simulink library "Engine_Lib"  (R2025a)
settings: Solver=ode45  StartTime=0.0  StopTime=10.0  RelTol=1e-3  EnableMultiTasking=on
undefined symbols (not defined in the file or in its folder): AFR_Table, beta, center, coeffs, DCT_Param, ECP_Table, exponent, ICP_Table, invDG, Load_Table, numterms, polyTerms, S_Table, WendlandNumTerms, width
libraries: fl_lib x8, nesl_utility x6, sdl_lib x1
(part 1 of 2)
Description:
  | Copyright 2014-2025 The MathWorks, Inc.
settings Model: Creator=smiller  LastModifiedBy=smiller
settings SolverCC: AlgebraicLoopSolver=TrustRegion
settings DataIOCC: LimitDataPoints=on  SaveFormat=Array  SignalLoggingSaveFormat=ModelDataLogs  ReturnWorkspaceOutputs=off
settings OptimizationCC: ReuseModelBlockBuffer=off  ExpressionDepthLimit=2147483647.0  LifeSpan=inf
settings DebuggingCC: UnderspecifiedInitializationDetection=Classic  MergeDetectMultiDrivingBlocksExec=none  SolverPrmCheckMsg=warning  FcnCallInpInsideContextMsg=warning  UnconnectedInputMsg=warning  UnconnectedOutputMsg=warning  UnconnectedLineMsg=warning  AllowSymbolicDim=off  StateNameClashWarn=warning  PregeneratedLibrarySubsystemCodeDiagnostic=none  SFUnexpectedBacktrackingDiag=warning  SFNoUnconditionalDefaultTransitionDiag=warning  SFExecutionAtInitializationDiag=none  ArithmeticOperatorsInVariantConditions=warning
settings HardwareCC: ProdBitPerPointer=32.0  ProdBitPerSizeT=32.0  ProdBitPerPtrDiffT=32.0  ProdLargestAtomicFloat=None  ProdIntDivRoundTo=Undefined  ProdEndianess=Unspecified  ProdWordSize=32.0  ProdHWDeviceType=32-bit Generic
settings ModelReferenceCC: EnableRefExpFcnMdlSchedulingChecks=on  PropagateSignalLabelsOutOfModel=off
settings SFSimCC: SimUseLocalCustomCode=off  CustomCodeUndefinedFunction=UseInterfaceOnly
settings RTWCC: RTWUseLocalCustomCode=off  GPUComputeCapability=3.5  DLArmComputeVersion=19.05
settings CodeAppCC: StateflowObjectComments=on
settings GRTTargetCC: TargetLangStandard=C89/C90 (ANSI)  CombineOutputUpdateFcns=off  GRTInterface=on
settings ConfigComp: CovMetricSettings=dw  CovSaveCumulativeToWorkspaceVar=on  CovSaveSingleToWorkspaceVar=on  CovExternalEMLEnable=off  CovSFcnEnable=off

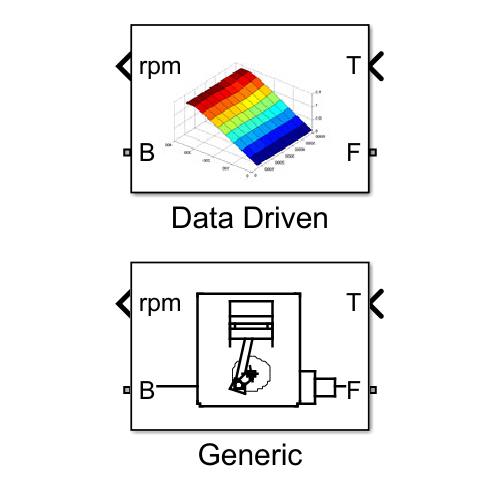
[thumbnail: Simulink's stored preview of the top-level diagram]
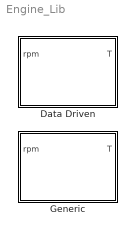
== system Engine_Lib ==
  Data Driven : Subsystem
      mask Display: image(imread('DCT_Engine_Data_Driven_IMAGE.jpg'));
  Generic : Subsystem
      mask Display:
      | plot([200.294537656123;201.704177092068;202.879954177142;203.81054553527;204.486989062962;204.902770239264;205.053884864158;204.938877621199;204.558856093007;203.917480094638;203.02092642757;201.877829393721;200.499197642409;198.898308151034;197.090578360535;195.093417696999;192.926059909376;191.349221415216], [79.0962651705123;81.4129472419303;83.856642682368;86.4038173688741;89.0299406167901;91.7097214236537;94.4173520353776;97.1267564890293;99.8118417386092;102.446748945347;105.006102512455;107.465254465996;109.80052182835;111.989414698229;114.010852840726;115.845368701499;117.475294889959;118.468271604945])
      | plot([180.070315486255;177.215173525063;174.340173090774;171.473002009205;168.641272705228;165.872256280019;163.192619875453;160.628169854943;158.203603274058;155.942270034374;153.865948011161;151.994633320535;150.346347745932;148.936965178479;147.780058742747;146.886770080143;146.265702048809;145.922835873396;145.861473542603;146.08220600922;146.58290749893;147.358755982674;148.402279615432;149.703428694174;151.249672441989;153.026119686324;155.015662269112;157.199139807684;159.555524219735;162.062122235246;164.694793945081;167.42818528151;170.23597219174;173.091114152932;175.966114587221;178.83328566879;181.665014972767;184.434031397976;185.486929355725], [123.25590763568;123.598773811093;123.660136141886;123.439403675268;122.938702185559;122.162853701815;121.119330069056;119.818180990315;118.2719372425;116.495489998164;114.505947415377;112.322469876805;109.966085464754;107.459487449243;104.826815739408;102.093424402979;99.2856374927491;96.4304955315569;93.5554950972677;90.688324015699;87.8565947117214;85.0875782865128;82.4079418819464;79.8434918614364;77.4189252805513;75.1575920408679;73.081270017655;71.2099553270291;69.5616697524256;68.1522871849724;66.9953807492411;66.1020920866371;65.4810240553025;65.1381578798894;65.0767955490969;65.2975280157144;65.7982295054238;66.5740779891678;66.9481130562871])
      | plot([182.088349247351;182.056804583223;181.962474383197;181.806267098667;181.589687091173;181.314820144583;180.98431337785;180.601349751811;180.169617415534;179.693274187426;179.176907513169;178.625490286111;178.044332955585;177.439032384376;176.815417947876;176.17949539401;175.537389004603;174.895282615196;174.25936006133;173.63574562483;173.030445053621;172.449287723095;171.897870496037;171.38150382178;170.905160593672;170.473428257395;170.090464631356;169.759957864623;169.485090918033;169.268510910539;169.112303626009;169.017973425983;168.986428761855;169.017973425983;169.112303626009;169.268510910539;169.485090918033;169.759957864623;170.090464631356;170.473428257395;170.905160593672;171.38150382178;171.897870496037;172.449287723095;173.030445053621;173.63574562483;174.25936006133;174.895282615196;175.537389004603;176.17949539401;176.815417947876;177.439032384376;178.044332955585;178.625490286111;179.176907513169;179.693274187426;180.169617415534;180.601349751811;180.98431337785;181.314820144583;181.589687091173;181.806267098667;181.962474383197;182.056804583223;182.088349247351;182.088349247351], [94.3432759959251;93.7073437064164;93.0775357924916;92.4599176486499;91.8604372752408;91.2848679959696;90.7387528576339;90.2273512475527;89.7555882427917;89.3280071789786;88.9487258954975;88.6213970784445;88.3491730832641;88.1346755758426;87.9799702844327;87.8865471055612;87.8553057555109;87.8865471055612;87.9799702844327;88.1346755758426;88.3491730832641;88.6213970784445;88.9487258954975;89.3280071789786;89.7555882427917;90.2273512475527;90.7387528576339;91.2848679959696;91.8604372752408;92.4599176486499;93.0775357924916;93.7073437064164;94.3432759959251;94.9792082854337;95.6090161993586;96.2266343432003;96.8261147166093;97.4016839958805;97.9477991342162;98.4592007442974;98.9309637490584;99.3585448128716;99.7378260963527;100.065154913406;100.337378908586;100.551876416008;100.706581707417;100.800004886289;100.831246236339;100.800004886289;100.706581707417;100.551876416008;100.337378908586;100.065154913406;99.7378260963526;99.3585448128716;98.9309637490584;98.4592007442974;97.9477991342162;97.4016839958805;96.8261147166093;96.2266343432003;95.6090161993586;94.9792082854338;94.3432759959251;94.3432759959251])
      | plot([201.615249970928;201.583705306799;201.489375106774;201.333167822243;201.11658781475;200.84172086816;200.511214101427;200.128250475388;199.69651813911;199.220174911002;198.703808236745;198.152391009688;197.571233679162;196.965933107953;196.342318671452;195.706396117586;195.06428972818;194.422183338773;193.786260784907;193.162646348407;192.557345777197;191.976188446671;191.424771219614;190.908404545357;190.432061317249;190.000328980971;189.617365354932;189.286858588199;189.011991641609;188.795411634116;188.639204349585;188.54487414956;188.513329485431;188.54487414956;188.639204349585;188.795411634116;189.011991641609;189.286858588199;189.617365354932;190.000328980971;190.432061317249;190.908404545357;191.424771219614;191.976188446671;192.557345777197;193.162646348407;193.786260784907;194.422183338773;195.06428972818;195.706396117586;196.342318671452;196.965933107953;197.571233679162;198.152391009688;198.703808236745;199.220174911002;199.69651813911;200.128250475388;200.511214101427;200.84172086816;201.11658781475;201.333167822243;201.489375106774;201.583705306799;201.615249970928;201.615249970928], [74.7533852700144;74.1174529805057;73.487645066581;72.8700269227392;72.2705465493302;71.694977270059;71.1488621317233;70.6374605216421;70.165697516881;69.7381164530679;69.3588351695868;69.0315063525339;68.7592823573535;68.5447848499319;68.390079558522;68.2966563796505;68.2654150296003;68.2966563796505;68.390079558522;68.5447848499319;68.7592823573535;69.0315063525339;69.3588351695868;69.7381164530679;70.165697516881;70.6374605216421;71.1488621317233;71.694977270059;72.2705465493302;72.8700269227392;73.487645066581;74.1174529805057;74.7533852700144;75.3893175595231;76.0191254734479;76.6367436172896;77.2362239906986;77.8117932699698;78.3579084083055;78.8693100183867;79.3410730231478;79.7686540869609;80.147935370442;80.4752641874949;80.7474881826754;80.9619856900969;81.1166909815068;81.2101141603783;81.2413555104285;81.2101141603783;81.1166909815068;80.9619856900969;80.7474881826753;80.4752641874949;80.147935370442;79.7686540869609;79.3410730231478;78.8693100183867;78.3579084083055;77.8117932699698;77.2362239906986;76.6367436172896;76.0191254734479;75.3893175595231;74.7533852700145;74.7533852700144])
      | plot([201.615249970928;201.583705306799;201.489375106774;201.333167822243;201.11658781475;200.84172086816;200.511214101427;200.128250475388;199.69651813911;199.220174911002;198.703808236745;198.152391009688;197.571233679162;196.965933107953;196.342318671452;195.706396117586;195.06428972818;194.422183338773;193.786260784907;193.162646348407;192.557345777197;191.976188446671;191.424771219614;190.908404545357;190.432061317249;190.000328980971;189.617365354932;189.286858588199;189.011991641609;188.795411634116;188.639204349585;188.54487414956;188.513329485431;188.54487414956;188.639204349585;188.795411634116;189.011991641609;189.286858588199;189.617365354932;190.000328980971;190.432061317249;190.908404545357;191.424771219614;191.976188446671;192.557345777197;193.162646348407;193.786260784907;194.422183338773;195.06428972818;195.706396117586;196.342318671452;196.965933107953;197.571233679162;198.152391009688;198.703808236745;199.220174911002;199.69651813911;200.128250475388;200.511214101427;200.84172086816;201.11658781475;201.333167822243;201.489375106774;201.583705306799;201.615249970928;201.615249970928], [74.7533852700144;74.1174529805057;73.487645066581;72.8700269227392;72.2705465493302;71.694977270059;71.1488621317233;70.6374605216421;70.165697516881;69.7381164530679;69.3588351695868;69.0315063525339;68.7592823573535;68.5447848499319;68.390079558522;68.2966563796505;68.2654150296003;68.2966563796505;68.390079558522;68.5447848499319;68.7592823573535;69.0315063525339;69.3588351695868;69.7381164530679;70.165697516881;70.6374605216421;71.1488621317233;71.694977270059;72.2705465493302;72.8700269227392;73.487645066581;74.1174529805057;74.7533852700144;75.3893175595231;76.0191254734479;76.6367436172896;77.2362239906986;77.8117932699698;78.3579084083055;78.8693100183867;79.3410730231478;79.7686540869609;80.147935370442;80.4752641874949;80.7474881826754;80.9619856900969;81.1166909815068;81.2101141603783;81.2413555104285;81.2101141603783;81.1166909815068;80.9619856900969;80.7474881826753;80.4752641874949;80.147935370442;79.7686540869609;79.3410730231478;78.8693100183867;78.3579084083055;77.8117932699698;77.2362239906986;76.6367436172896;76.0191254734479;75.3893175595231;74.7533852700145;74.7533852700144])
      | plot([142.90856779553;142.90856779553;208.103220211342;208.103220211342], [139.948037685826;218.181620584801;218.181620584801;139.948037685826])
      | plot([142.90856779553;208.103220211342], [179.064829135314;179.064829135314])
      | plot([149.459528038278;149.459528038278], [179.064829135314;172.576858894899])
      | plot([201.615249970928;201.615249970928], [179.064829135314;172.576858894899])
      | plot([142.90856779553;208.103220211342;208.103220211342;142.90856779553;142.90856779553], [179.064829135314;179.064829135314;152.986968168989;152.986968168989;179.064829135314])
      | plot([142.90856779553;208.103220211342], [192.103759618476;192.103759618476])
      | plot([180.639579193667;200.229469919577], [99.0045361686498;79.4776354450732])
      | plot([173.332738922909;192.92262964882], [87.8553057555109;68.3284050319344])
      | plot([183.663099305704;200.481429928914], [153.553878189996;76.9580353517085])
      | plot([184.544959338382;174.970478983596], [95.0361660216004;153.553878189996])
      | plot([183.474129298702;186.749609420076;206.654450157657;201.615249970928;197.961829835549], [76.9580353517085;62.0923948008567;67.8874750155956;88.1702557671815;87.7923157531768])
      | plot([164.199188584462;187.694459455088], [94.7842060122639;95.1621460262686])
      | plot([175.537389004603;175.285428995267], [106.50034644641;81.9342455361038])
      | plot([142.90856779553;208.103220211342], [172.576858894899;172.576858894899])
      | plot([255.86397353746;317.389525743201], [71.0999651346356;71.0999651346356])
      | plot([80.518472487107;50.86397353746;50.86397353746;80.518472487107;80.518472487107], [85.2727156598121;85.2727156598121;56.927214609459;56.927214609459;85.2727156598121])
      | plot([102.180272066966;80.518472487107;80.518472487107;102.180272066966], [42.7544640842825;42.7544640842825;99.4454661849886;99.4454661849886])
      | plot([108.893966535106;108.245686045801;107.603648851995;106.974038122836;106.362917353826;105.776171972045;105.219452656266;104.698120917834;104.217197466378;103.781313857637;103.394667889039;103.060983172626;102.783473274627;102.564810767061;102.40710148941;102.31186426823;102.280016290024;102.280016290024;102.31186426823;102.40710148941;102.564810767061;102.783473274627;103.060983172626;103.394667889039;103.781313857637;104.217197466378;104.698120917834;105.219452656266;105.776171972045;106.362917353826;106.974038122836;107.603648851995;108.245686045801;108.893966535106;249.67662175186;250.324902241165;250.966939434972;251.596550164131;252.20767093314;252.794416314921;253.3511356307;253.872467369133;254.353390820588;254.78927442933;255.175920397927;255.50960511434;255.787115012339;256.005777519905;256.163486797556;256.258724018736;256.290571996942;256.290571996942;256.258724018736;256.163486797556;256.005777519905;255.787115012339;255.50960511434;255.175920397927;254.78927442933;254.353390820588;253.872467369133;253.3511356307;252.794416314921;252.20767093314;251.596550164131;250.966939434972;250.324902241165;249.67662175186;108.893966535106], [233.173241140321;233.141393162114;233.046155940935;232.888446663284;232.669784155718;232.392274257719;232.058589541306;231.671943572708;231.236059963967;230.755136512511;230.233804774079;229.6770854583;229.090340076519;228.479219307509;227.84960857835;227.207571384544;226.559290895239;46.5338642243296;45.8855837350246;45.2435465412178;44.6139358120588;44.0028150430496;43.4160696612682;42.8593503454891;42.3380186070568;41.8570951556014;41.4212115468599;41.0345655782626;40.7008808618494;40.42337096385;40.2047084562844;40.0469991786335;39.9517619574538;39.9199139792472;39.9199139792472;39.9517619574538;40.0469991786335;40.2047084562844;40.42337096385;40.7008808618494;41.0345655782626;41.4212115468599;41.8570951556014;42.3380186070568;42.8593503454891;43.4160696612682;44.0028150430496;44.6139358120588;45.2435465412178;45.8855837350246;46.5338642243296;226.559290895239;227.207571384544;227.84960857835;228.479219307509;229.090340076519;229.6770854583;230.233804774079;230.755136512511;231.236059963967;231.671943572708;232.058589541306;232.392274257719;232.669784155718;232.888446663284;233.046155940935;233.141393162114;233.173241140321;233.173241140321])
      | plot([50.280016290024;35.236212508752942], [71.0999651346356;71.0999651346356]);
      | patch([0;354.791188146919;354.791188146919;0;0;0.472425017505884;0.472425017505884;354.318763129413;354.318763129413;0.472425017505884;0], [283.927435521036;283.927435521036;0;0;283.927435521036;283.455010503531;0.472425017505884;0.472425017505884;283.455010503531;283.455010503531;283.927435521036], [1;1;1])

== system Engine_Lib/Data Driven ==
  T : Inport
  Engine Control Software : Subsystem
  Inertia : fl_lib/Mechanical/Rotational Elements/Inertia  inertia=DCT_Param.ICE.Shaft_Inertia kg*m^2  num_ports=foundation.enum.numPorts2.one  w_specify=on  w_priority=High  w=DCT_Param.ICE.Initial_Velocity rpm  w_nominal_specify=off  w_nominal_value=1  w_nominal_unit=rad/s  t_specify=off  t_priority=High  t=0 N*m  t_nominal_specify=off  t_nominal_value=1  t_nominal_unit=N*m
  MBC Engine Model From Dynamometer Data : Subsystem
      mask Display:
      | image(imread('DCT_Engine_Data_Driven_IMAGE.jpg'),'center')
      | port_label('input',1,'Bus')
      | port_label('output',1,'rpm')
      | color('red');
      | port_label('LConn',1,'B')
      | port_label('RConn',1,'F')
  B : PMIOPort  Side=Right
  F : PMIOPort  Port=2  Side=Left
  rpm : Outport  VectorParamsAs1DForOutWhenUnconnected=off
  wires:
  Engine Control Software/1(Engine Control Bus) -> MBC Engine Model From Dynamometer Data/1(Engine Control Bus)
  MBC Engine Model From Dynamometer Data/1(Engine Speed) -> Engine Control Software/1(Engine Speed), rpm/1
  T/1 -> Engine Control Software/2(Torque Demand)
  connections:
  B/RConn1 -- MBC Engine Model From Dynamometer Data/LConn1
  F/RConn1 -- MBC Engine Model From Dynamometer Data/RConn1 -- Inertia/LConn1

== system Engine_Lib/Generic ==
  T : Inport
  Engine Management : Subsystem
  Fuel Consumption : Subsystem
  Generic Engine : sdl_lib/Engines & Motors/Generic Engine  input_type=sdl.enum.GenericEngineInputType.NormalizedThrottle  model_parameterization=1  engine_type=1  Trq_max=380 N*m  w_Trq_max=4300 rpm  P_max=DCT_Param.ICE.Max_Power W  w_P_max=DCT_Param.ICE.Speed_At_Max_Power rpm  w_max=DCT_Param.ICE.Max_Speed rpm  w_min=DCT_Param.ICE.Stall_Speed rpm  w_tab=[ 500 1000 2e+3 3e+3 4e+3 5e+3 6e+3 7e+3 ] rpm  trq_tab=[ 380 380 380 380 350 280 200 80 ] N*m  pwr_tab=[ 2e+4 4e+4 7.8e+4 1.2e+5 1.45e+5 1.48e+5 1.25e+5 6e+4 ] W  interp_method=1  w_thr=DCT_Param.ICE.Speed_Threshold rpm  model_inertia=1  inertia=DCT_Param.ICE.Shaft_Inertia kg*m^2  initial_velocity=DCT_Param.ICE.Initial_Velocity rpm  model_time_constant=1  time_constant=DCT_Param.ICE.Engine_Time_Constant s  initial_normalized_throttle=DCT_Param.ICE.Initial_Normalized_Throttle  fc_model=1  fc_per_rev=25 mg/rev  fc_w_tab=[ 1000 2e+3 3e+3 4e+3 5e+3 6e+3 ] rpm  fc_trq_tab=[ 0 80 160 200 240 320 360 400 ] N*m  fc_tab=[ 0.5 0.9 1.4 1.6 1.9 2.7 3.4 4.4; 1 1.7 2.7 3.1 3.6 5 6 7.4; 1.4 2.7 4 4.8 5.6 7.5 8.5 10.5; 2 3.6 5.8 6.7 8 10.4 11.7 13.3; 2.5 4.8 7.9 9.4 10.8 14 16.2 18.6; 3.1 6 10.3 11.9 13.8 18.4 22 26.5 ] g/s  bmep_tab=[ 0 250 500 625 750 1000 1.15e+3 1.25e+3 ] kPa  bsfc_tab=[ 410 380 300 280 270 290 320 380; 410 370 290 270 260 270 285 320; 415 380 290 275 265 270 270 300; 420 390 310 290 285 280 280 285; 430 410 340 320 310 300 310 320; 450 430 370 340 330 330 350 380 ] g/hr/kW  fc_interp_method=1  displaced_volume=400 cm^3  rev_per_cycle=2  idle_speed=0  idle_speed_reference=1000 rpm  tau_controller=1 s  idle_w_thr=1 rpm  redline=0  redline_speed=5000 rpm  tau_redline=1 s  redline_w_thr=1 rpm
      settings: InternalSimscapePortConfiguration="{\"Bottom\":[],\"Left\":[{\"id\":\"ThrNorm\",\"label\":\"Thr\",\"type\":\"input\"},{\"id\":\"B\",\"label\":\"B\",\"type\":\"foundation.mechanical.rotational.rotational\"}],\"Right\":[{\"id\":\"P\",\"label\":\"P\",\"type\":\"output\"},{\"id\":\"FC\",\"label\":\"FC\",\"type\":\"output\"},{\"id\":\"F\",\"label\":\"F\",\"type\":\"foundation.mechanical.rotational.rotational\"}],\"Top\":[]}"
  F : PMIOPort  Side=Left
  B : PMIOPort  Port=2  Side=Right
  rpm : Outport  VectorParamsAs1DForOutWhenUnconnected=off
  wires:
  T/1 -> Engine Management/2(TrqDem)
  Fuel Consumption/1(rpm) -> rpm/1, Engine Management/1(EngSpd)
  connections:
  B/RConn1 -- Generic Engine/LConn2
  Engine Management/RConn1 -- Generic Engine/LConn1
  Generic Engine/RConn3 -- Fuel Consumption/LConn1
  Fuel Consumption/RConn1 -- F/RConn1

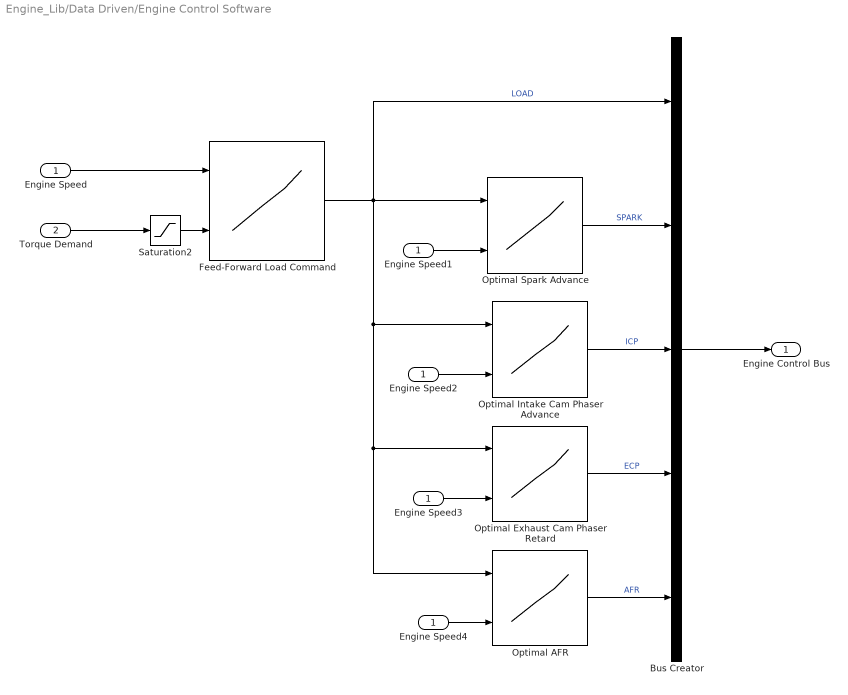
== system Engine_Lib/Data Driven/Engine Control Software ==
  Engine Speed : Inport
  Torque Demand : Inport  Port=2
  Bus Creator : BusCreator  Inputs=5
  Engine Speed{1..4} (4 alike) : InportShadow
  Feed-Forward Load Command : Lookup2D  RowIndex=Load_Table.Y  ColumnIndex=Load_Table.X  Table=Load_Table.Z  LookUpMeth=Interpolation-Use End Values  SaturateOnIntegerOverflow=off  InputSameDT=off
  Optimal AFR : Lookup2D  RowIndex=AFR_Table.Y  ColumnIndex=AFR_Table.X  Table=AFR_Table.Z  LookUpMeth=Interpolation-Use End Values  SaturateOnIntegerOverflow=off  InputSameDT=off
  Optimal Exhaust Cam Phaser Retard : Lookup2D  RowIndex=ECP_Table.Y  ColumnIndex=ECP_Table.X  Table=ECP_Table.Z  LookUpMeth=Interpolation-Use End Values  SaturateOnIntegerOverflow=off  InputSameDT=off
  Optimal Intake Cam Phaser Advance : Lookup2D  RowIndex=ICP_Table.Y  ColumnIndex=ICP_Table.X  Table=ICP_Table.Z  LookUpMeth=Interpolation-Use End Values  SaturateOnIntegerOverflow=off  InputSameDT=off
  Optimal Spark Advance : Lookup2D  RowIndex=S_Table.Y  ColumnIndex=S_Table.X  Table=S_Table.Z  LookUpMeth=Interpolation-Use End Values  SaturateOnIntegerOverflow=off  InputSameDT=off
  Saturation2 : Saturate  UpperLimit=inf  LowerLimit=0
  Engine Control Bus : Outport  VectorParamsAs1DForOutWhenUnconnected=off
  wires:
  Torque Demand/1 -> Saturation2/1
  Engine Speed/1 -> Feed-Forward Load Command/1
  Optimal Spark Advance/1 -> Bus Creator/2  "SPARK"
  Optimal Intake Cam Phaser Advance/1 -> Bus Creator/3  "ICP"
  Optimal Exhaust Cam Phaser Retard/1 -> Bus Creator/4  "ECP"
  Optimal AFR/1 -> Bus Creator/5  "AFR"
  Bus Creator/1 -> Engine Control Bus/1
  Engine Speed4/1 -> Optimal AFR/2
  Engine Speed3/1 -> Optimal Exhaust Cam Phaser Retard/2
  Engine Speed2/1 -> Optimal Intake Cam Phaser Advance/2
  Engine Speed1/1 -> Optimal Spark Advance/2
  Feed-Forward Load Command/1 -> Optimal Spark Advance/1, Optimal Intake Cam Phaser Advance/1, Optimal Exhaust Cam Phaser Retard/1, Optimal AFR/1, Bus Creator/1  "LOAD"
  Saturation2/1 -> Feed-Forward Load Command/2

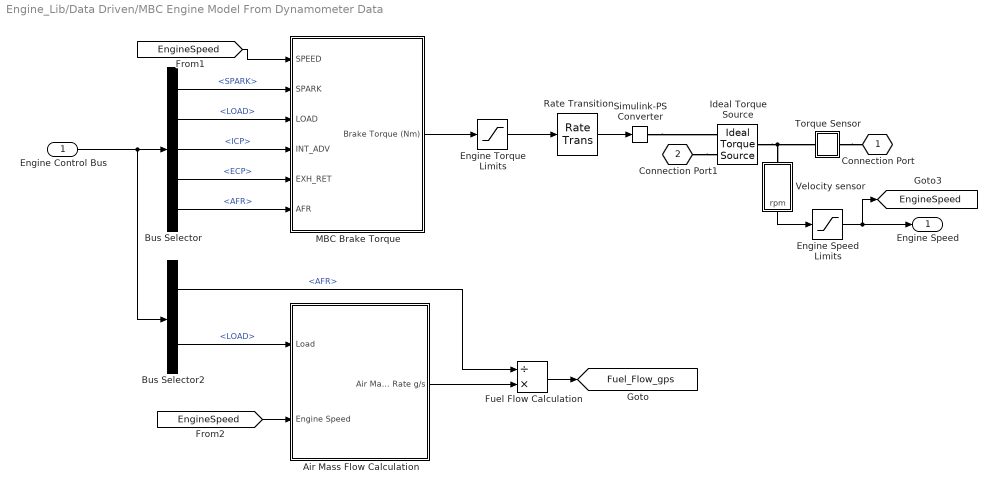
== system Engine_Lib/Data Driven/MBC Engine Model From Dynamometer Data ==
  Engine Control Bus : Inport
  Air Mass Flow Calculation : Subsystem
  Bus Selector : BusSelector  OutputSignals=SPARK,LOAD,ICP,ECP,AFR
  Bus Selector2 : BusSelector  OutputSignals=AFR,LOAD
  Engine Speed Limits : Saturate  UpperLimit=inf  LowerLimit=500
  Engine Torque Limits : Saturate  UpperLimit=Inf  LowerLimit=0.1
  Fuel Flow Calculation : Product  Inputs=/*  RndMeth=Zero
  Ideal Torque Source : fl_lib/Mechanical/Mechanical Sources/Ideal Torque Source
  MBC Brake Torque : Subsystem
  Rate Transition : RateTransition
  Simulink-PS Converter : nesl_utility/Simulink-PS Converter  PhysicalDomain=network_engine_domain  SubClassName=ps_input  LeftPortType=input  RightPortType=output  PseudoPeriodic=off  Frequencies=[]  NoiseDistribution=none  NoiseParameters=[]  Unit=1  AffineConversion=off  FilteringAndDerivatives=zero  SimscapeFilterOrder=1  InputFilterTimeConstant=0.005  UdotUserProvided=0
  Torque Sensor : Subsystem
      mask Display: disp('S')
  Velocity sensor : Subsystem
  Connection Port : PMIOPort  Side=Right
  Connection Port1 : PMIOPort  Port=2  Side=Left
  Engine Speed : Outport  VectorParamsAs1DForOutWhenUnconnected=off
  tag scope: EngineSpeed=global, Fuel_Flow_gps=global
  wires:
  Engine Torque Limits/1 -> Rate Transition/1
  Bus Selector2/2 -> Air Mass Flow Calculation/1(Load)  "<LOAD>"
  Bus Selector2/1 -> Fuel Flow Calculation/1  "<AFR>"
  Air Mass Flow Calculation/1(Air Mass Flow Rate g/s) -> Fuel Flow Calculation/2
  [EngineSpeed] -> Air Mass Flow Calculation/2(Engine Speed)
  Fuel Flow Calculation/1 -> [Fuel_Flow_gps]
  MBC Brake Torque/1(Brake Torque (Nm)) -> Engine Torque Limits/1
  Engine Control Bus/1 -> Bus Selector2/1, Bus Selector/1
  Rate Transition/1 -> Simulink-PS Converter/1
  Velocity sensor/1(rpm) -> Engine Speed Limits/1
  Engine Speed Limits/1 -> Engine Speed/1, [EngineSpeed]
  [EngineSpeed] -> MBC Brake Torque/1(SPEED)
  Bus Selector/1 -> MBC Brake Torque/2(SPARK)  "<SPARK>"
  Bus Selector/2 -> MBC Brake Torque/3(LOAD)  "<LOAD>"
  Bus Selector/3 -> MBC Brake Torque/4(INT_ADV)  "<ICP>"
  Bus Selector/4 -> MBC Brake Torque/5(EXH_RET)  "<ECP>"
  Bus Selector/5 -> MBC Brake Torque/6(AFR)  "<AFR>"
  connections:
  Ideal Torque Source/LConn1 -- Velocity sensor/LConn1 -- Torque Sensor/LConn1
  Connection Port1/RConn1 -- Ideal Torque Source/RConn2
  Simulink-PS Converter/RConn1 -- Ideal Torque Source/RConn1
  Torque Sensor/RConn1 -- Connection Port/RConn1

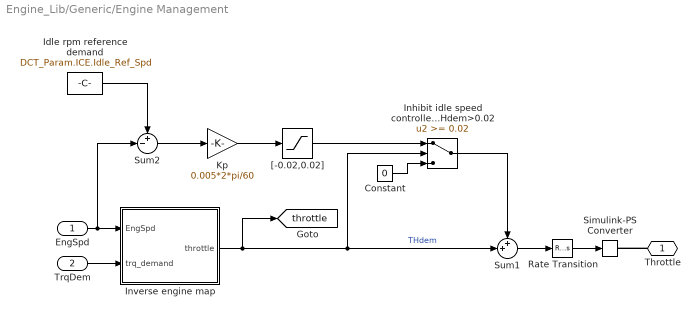
== system Engine_Lib/Generic/Engine Management ==
  EngSpd : Inport
  TrqDem : Inport  Port=2
  Constant : Constant  Value=0  SampleTime=0.01
  Idle rpm reference demand : Constant  Value=DCT_Param.ICE.Idle_Ref_Spd  SampleTime=0.01
  Inhibit idle speed controller if THdem>0.02 : Switch  Threshold=0.02  SaturateOnIntegerOverflow=off
  Inverse engine map : Subsystem  mask(Inverse engine map){P0=92000, rpm0=5500}
      mask prompts: P0 "Engine maximum power (W)"; rpm0 "Speed at maximum power (rpm)"
      mask help: Converts measured speed and demanded torque into normalized throttle demand. Assumes that the engine is modeled using the Simscape Driveline Generic Engine block with model parameterization set to Normalized 3rd-order polynomial matched to peak power.
      mask init:
      | w0 = 2*pi*rpm0/60;
  Kp : Gain  Gain=0.005*2*pi/60  SaturateOnIntegerOverflow=on  OutDataTypeStr=Inherit: Same as input  ParamDataTypeStr=Inherit: Same as input
  Rate Transition : RateTransition
  Simulink-PS Converter : nesl_utility/Simulink-PS Converter  PhysicalDomain=network_engine_domain  SubClassName=ps_input  LeftPortType=input  RightPortType=output  PseudoPeriodic=off  Frequencies=[]  NoiseDistribution=none  NoiseParameters=[]  Unit=1  AffineConversion=off  FilteringAndDerivatives=zero  SimscapeFilterOrder=1  InputFilterTimeConstant=0.005  UdotUserProvided=0
  Sum1 : Sum  Inputs=++|  InputSameDT=on  SaturateOnIntegerOverflow=on  OutDataTypeStr=Inherit: Same as first input
  Sum2 : Sum  Inputs=+-|  InputSameDT=on  SaturateOnIntegerOverflow=on  OutDataTypeStr=Inherit: Same as first input
  "[-0.02,0.02]" : Saturate  UpperLimit=0.02  LowerLimit=-0.02
  Throttle : PMIOPort  Side=Right
  tag scope: throttle=global
  wires:
  "[-0.02,0.02]"/1 -> Inhibit idle speed controller if THdem>0.02/1
  Kp/1 -> "[-0.02,0.02]"/1
  Sum2/1 -> Kp/1
  Idle rpm reference demand/1 -> Sum2/1
  Sum1/1 -> Rate Transition/1
  Constant/1 -> Inhibit idle speed controller if THdem>0.02/3
  Inhibit idle speed controller if THdem>0.02/1 -> Sum1/1
  EngSpd/1 -> Sum2/2, Inverse engine map/1(EngSpd)
  TrqDem/1 -> Inverse engine map/2(trq_demand)
  Inverse engine map/1(throttle) -> Inhibit idle speed controller if THdem>0.02/2, Sum1/2, [throttle]  "THdem"
  Rate Transition/1 -> Simulink-PS Converter/1
  connections:
  Throttle/RConn1 -- Simulink-PS Converter/RConn1

== system Engine_Lib/Generic/Fuel Consumption ==
  Filter : TransferFcn  Denominator=[DCT_Param.Transmission.Abstract.Ratio_Time_Const*2 1]
  Fuel Consumption Table : Lookup2D  RowIndex=DCT_Param.ICE.FC.Speed_Vector  ColumnIndex=DCT_Param.ICE.FC.Torque_Vector  Table=DCT_Param.ICE.FC.Consumption_Table  SaturateOnIntegerOverflow=off  InputSameDT=off
  Min of table : Saturate  UpperLimit=Inf  LowerLimit=min(min(DCT_Param.ICE.FC.Consumption_Table))
  Torque Sensor : Subsystem
      mask Display: disp('S')
  Velocity sensor : Subsystem
      mask Display: disp('S')
  B : PMIOPort  Side=Left
  F : PMIOPort  Port=2  Side=Right
  rpm : Outport  VectorParamsAs1DForOutWhenUnconnected=off
  tag scope: Fuel_Flow_gps=global
  wires:
  Velocity sensor/1(rpm) -> rpm/1, Fuel Consumption Table/1
  Fuel Consumption Table/1 -> Min of table/1
  Torque Sensor/1(rpm) -> Filter/1
  Filter/1 -> Fuel Consumption Table/2
  Min of table/1 -> [Fuel_Flow_gps]
  connections:
  B/RConn1 -- Torque Sensor/LConn1 -- Velocity sensor/LConn1
  Torque Sensor/RConn1 -- F/RConn1

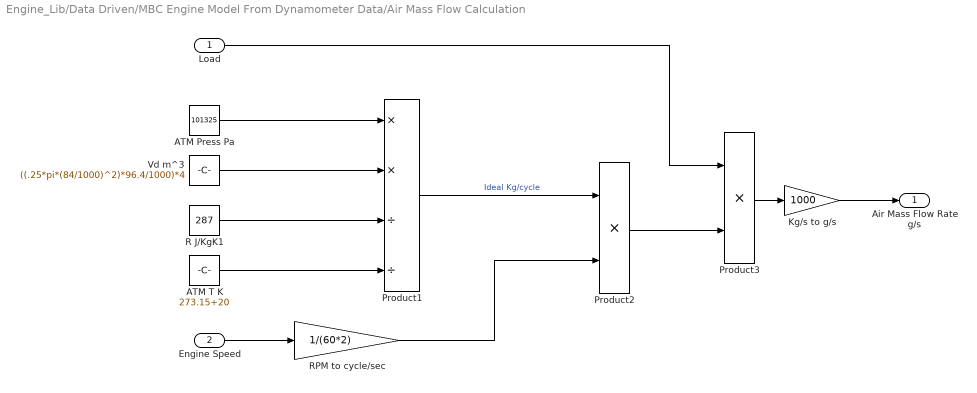
== system Engine_Lib/Data Driven/MBC Engine Model From Dynamometer Data/Air Mass Flow Calculation ==
  Load : Inport
  Engine Speed : Inport  Port=2
  ATM Press Pa : Constant  Value=101325
  ATM T K : Constant  Value=273.15+20
  Kg/s to g/s : Gain  Gain=1000
  Product1 : Product  Inputs=**//  InputSameDT=on  SaturateOnIntegerOverflow=on  OutDataTypeStr=Inherit: Same as first input
  Product2 : Product  Inputs=**  InputSameDT=on  SaturateOnIntegerOverflow=on  OutDataTypeStr=Inherit: Same as first input
  Product3 : Product  Inputs=**  InputSameDT=on  SaturateOnIntegerOverflow=on  OutDataTypeStr=Inherit: Same as first input
  R J/KgK1 : Constant  Value=287
  RPM to cycle/sec : Gain  Gain=1/(60*2)  SaturateOnIntegerOverflow=on  OutDataTypeStr=Inherit: Same as input  ParamDataTypeStr=Inherit: Same as input
  Vd m^3 : Constant  Value=((.25*pi*(84/1000)^2)*96.4/1000)*4
  Air Mass Flow Rate g/s : Outport  VectorParamsAs1DForOutWhenUnconnected=off
  wires:
  Kg/s to g/s/1 -> Air Mass Flow Rate g/s/1
  Product3/1 -> Kg/s to g/s/1
  Product2/1 -> Product3/2
  RPM to cycle/sec/1 -> Product2/2
  Engine Speed/1 -> RPM to cycle/sec/1
  Vd m^3/1 -> Product1/2
  ATM T K/1 -> Product1/4
  R J/KgK1/1 -> Product1/3
  ATM Press Pa/1 -> Product1/1
  Load/1 -> Product3/1
  Product1/1 -> Product2/1  "Ideal Kg/cycle"

== system Engine_Lib/Data Driven/MBC Engine Model From Dynamometer Data/MBC Brake Torque ==
  SPEED : Inport
  SPARK : Inport  Port=2
  LOAD : Inport  Port=3
  INT_ADV : Inport  Port=4
  EXH_RET : Inport  Port=5
  AFR : Inport  Port=6
  Mx1 : Mux  Inputs=6
  xregtwostage : Subsystem
  Brake Torque (Nm) : Outport  VectorParamsAs1DForOutWhenUnconnected=off
  wires:
  xregtwostage/1(Y) -> Brake Torque (Nm)/1
  Mx1/1 -> xregtwostage/1(X)
  AFR/1 -> Mx1/6
  EXH_RET/1 -> Mx1/5
  INT_ADV/1 -> Mx1/4
  LOAD/1 -> Mx1/3
  SPEED/1 -> Mx1/2
  SPARK/1 -> Mx1/1

== system Engine_Lib/Data Driven/MBC Engine Model From Dynamometer Data/Torque Sensor ==
  Ideal Torque Sensor : fl_lib/Mechanical/Mechanical Sensors/Ideal Torque Sensor
  PS-Simulink Converter1 : nesl_utility/PS-Simulink Converter  PhysicalDomain=network_engine_domain  SubClassName=ps_output  LeftPortType=input  RightPortType=output  PseudoPeriodic=off  Frequencies=[]  VectorFormat=1-D array  Unit=N*m  AffineConversion=off
  R : PMIOPort  Side=Left
  C : PMIOPort  Port=2  Side=Right
  tag scope: EngTrq_Nm=global
  wires:
  PS-Simulink Converter1/1 -> [EngTrq_Nm]
  connections:
  Ideal Torque Sensor/RConn2 -- PS-Simulink Converter1/LConn1
  C/RConn1 -- Ideal Torque Sensor/RConn1
  R/RConn1 -- Ideal Torque Sensor/LConn1

== system Engine_Lib/Data Driven/MBC Engine Model From Dynamometer Data/Velocity sensor ==
  Ideal Rotational Motion Sensor : fl_lib/Mechanical/Mechanical Sensors/Ideal Rotational Motion Sensor  reference=foundation.enum.MeasurementReference.difference  acceleration_port=false  velocity_port=true  position_port=true  wrap_angle=simscape.enum.onoff.off  offset=5 rad
  MRR : fl_lib/Mechanical/Rotational Elements/Mechanical Rotational Reference
  PS2S : nesl_utility/PS-Simulink Converter  PhysicalDomain=network_engine_domain  SubClassName=ps_output  LeftPortType=input  RightPortType=output  PseudoPeriodic=off  Frequencies=[]  VectorFormat=1-D array  Unit=rpm  AffineConversion=off
  Sensor dynamics : TransferFcn  Denominator=[0.01 1]
  Zero-Order Hold : ZeroOrderHold  SampleTime=0.01
  F : PMIOPort  Side=Left
  rpm : Outport  VectorParamsAs1DForOutWhenUnconnected=off
  wires:
  PS2S/1 -> Sensor dynamics/1
  Zero-Order Hold/1 -> rpm/1
  Sensor dynamics/1 -> Zero-Order Hold/1
  connections:
  F/RConn1 -- Ideal Rotational Motion Sensor/LConn1
  Ideal Rotational Motion Sensor/RConn2 -- PS2S/LConn1
  MRR/LConn1 -- Ideal Rotational Motion Sensor/RConn1

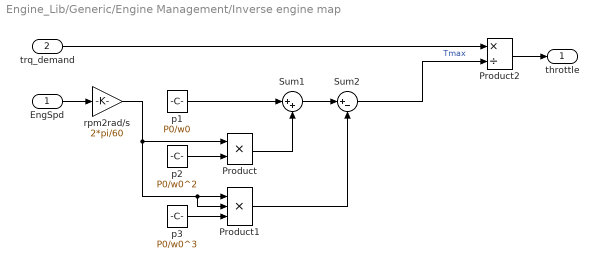
== system Engine_Lib/Generic/Engine Management/Inverse engine map ==
  EngSpd : Inport
  trq_demand : Inport  Port=2
  Product : Product  InputSameDT=on  SaturateOnIntegerOverflow=on  OutDataTypeStr=Inherit: Same as first input
  Product1 : Product  Inputs=3  InputSameDT=on  SaturateOnIntegerOverflow=on  OutDataTypeStr=Inherit: Same as first input
  Product2 : Product  Inputs=*/  InputSameDT=on  SaturateOnIntegerOverflow=on  OutDataTypeStr=Inherit: Same as first input
  Sum1 : Sum  Inputs=|++  InputSameDT=on  SaturateOnIntegerOverflow=on  OutDataTypeStr=Inherit: Same as first input
  Sum2 : Sum  Inputs=|+-  InputSameDT=on  SaturateOnIntegerOverflow=on  OutDataTypeStr=Inherit: Same as first input
  p1 : Constant  Value=P0/w0
  p2 : Constant  Value=P0/w0^2
  p3 : Constant  Value=P0/w0^3
  rpm2rad/s : Gain  Gain=2*pi/60  SaturateOnIntegerOverflow=on  OutDataTypeStr=Inherit: Same as input  ParamDataTypeStr=Inherit: Same as input
  throttle : Outport  VectorParamsAs1DForOutWhenUnconnected=off
  wires:
  EngSpd/1 -> rpm2rad/s/1
  trq_demand/1 -> Product2/1
  rpm2rad/s/1 -> Product/1, Product1/1, Product1/2
  p2/1 -> Product/2
  Product/1 -> Sum1/2
  p3/1 -> Product1/3
  Sum1/1 -> Sum2/1
  Product1/1 -> Sum2/2
  Product2/1 -> throttle/1
  Sum2/1 -> Product2/2  "Tmax"
  p1/1 -> Sum1/1

== system Engine_Lib/Generic/Fuel Consumption/Torque Sensor ==
  Ideal Torque Sensor : fl_lib/Mechanical/Mechanical Sensors/Ideal Torque Sensor
  PS-Simulink Converter1 : nesl_utility/PS-Simulink Converter  PhysicalDomain=network_engine_domain  SubClassName=ps_output  LeftPortType=input  RightPortType=output  PseudoPeriodic=off  Frequencies=[]  VectorFormat=1-D array  Unit=N*m  AffineConversion=off
  R : PMIOPort  Side=Left
  C : PMIOPort  Port=2  Side=Right
  rpm : Outport  VectorParamsAs1DForOutWhenUnconnected=off
  tag scope: EngTrq_Nm=global
  wires:
  PS-Simulink Converter1/1 -> [EngTrq_Nm], rpm/1
  connections:
  Ideal Torque Sensor/RConn2 -- PS-Simulink Converter1/LConn1
  C/RConn1 -- Ideal Torque Sensor/RConn1
  R/RConn1 -- Ideal Torque Sensor/LConn1

== system Engine_Lib/Generic/Fuel Consumption/Velocity sensor ==
  Ideal Rotational Motion Sensor : fl_lib/Mechanical/Mechanical Sensors/Ideal Rotational Motion Sensor  reference=foundation.enum.MeasurementReference.difference  acceleration_port=false  velocity_port=true  position_port=true  wrap_angle=simscape.enum.onoff.off  offset=0 rad
  MRR : fl_lib/Mechanical/Rotational Elements/Mechanical Rotational Reference
  PS2S : nesl_utility/PS-Simulink Converter  PhysicalDomain=network_engine_domain  SubClassName=ps_output  LeftPortType=input  RightPortType=output  PseudoPeriodic=off  Frequencies=[]  VectorFormat=1-D array  Unit=rpm  AffineConversion=off
  Sensor dynamics : TransferFcn  Denominator=[0.01 1]
  Zero-Order Hold : ZeroOrderHold  SampleTime=0.01
  F : PMIOPort  Side=Left
  rpm : Outport  VectorParamsAs1DForOutWhenUnconnected=off
  wires:
  Zero-Order Hold/1 -> rpm/1
  Sensor dynamics/1 -> Zero-Order Hold/1
  PS2S/1 -> Sensor dynamics/1
  connections:
  MRR/LConn1 -- Ideal Rotational Motion Sensor/RConn1
  Ideal Rotational Motion Sensor/RConn2 -- PS2S/LConn1
  F/RConn1 -- Ideal Rotational Motion Sensor/LConn1

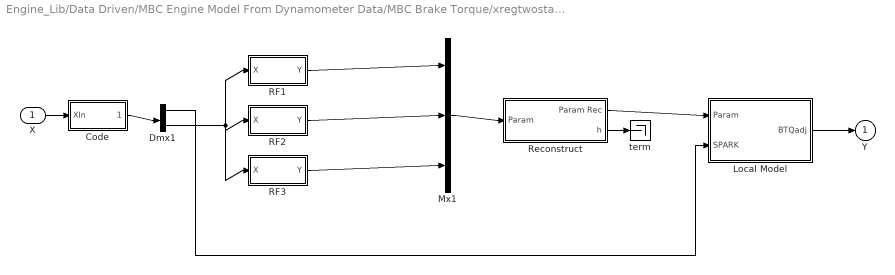
== system Engine_Lib/Data Driven/MBC Engine Model From Dynamometer Data/MBC Brake Torque/xregtwostage ==
  X : Inport
  Code : Subsystem
  Dmx1 : Demux  Outputs="[ 1  -1]"
      settings: DisplayOption=none
  Local Model : Subsystem
      mask init:
      | xregmaskinitialization;
  Mx1 : Mux  Inputs=3
  RF1 : Subsystem
      mask init:
      | xregmaskinitialization;
  RF2 : Subsystem
      mask init:
      | xregmaskinitialization;
  RF3 : Subsystem
      mask init:
      | xregmaskinitialization;
  Reconstruct : Subsystem
      mask init:
      | xregmaskinitialization;
  term : Terminator
  Y : Outport  VectorParamsAs1DForOutWhenUnconnected=off
  wires:
  Reconstruct/2(h) -> term/1
  Local Model/1(BTQadj) -> Y/1
  Reconstruct/1(Param Rec) -> Local Model/1(Param)
  Mx1/1 -> Reconstruct/1(Param)
  RF3/1(Y) -> Mx1/3
  RF2/1(Y) -> Mx1/2
  RF1/1(Y) -> Mx1/1
  Dmx1/1 -> Local Model/2(SPARK)
  Dmx1/2 -> RF3/1(X), RF2/1(X), RF1/1(X)
  Code/1(XCoded) -> Dmx1/1
  X/1 -> Code/1(XIn)

== system Engine_Lib/Data Driven/MBC Engine Model From Dynamometer Data/MBC Brake Torque/xregtwostage/Code ==
  XIn : Inport
  Mid : Constant  Value=[25 3255.40527503736 0.832989154540633 22.4723365216774 22.4387901165607 12.6 ]
  demux : Demux  Outputs=6
      settings: DisplayOption=none
  gain : Gain  Gain=[0.04 0.000372414635111356 1.57980884110427 0.0365584433472559 0.0365685104958011 0.434782608695652 ]  SaturateOnIntegerOverflow=on  OutDataTypeStr=Inherit: Same as input  ParamDataTypeStr=Inherit: Same as input
  mux : Mux  Inputs=6
  sum : Sum  Inputs=-+|  InputSameDT=on  SaturateOnIntegerOverflow=on  OutDataTypeStr=Inherit: Same as first input
  XCoded : Outport  VectorParamsAs1DForOutWhenUnconnected=off
  wires:
  gain/1 -> XCoded/1
  sum/1 -> gain/1
  mux/1 -> sum/2
  XIn/1 -> demux/1
  Mid/1 -> sum/1
  demux/6 -> mux/6
  demux/5 -> mux/5
  demux/4 -> mux/4
  demux/3 -> mux/3
  demux/2 -> mux/2
  demux/1 -> mux/1

== system Engine_Lib/Data Driven/MBC Engine Model From Dynamometer Data/MBC Brake Torque/xregtwostage/Local Model ==
  Param : Inport
  SPARK : Inport  Port=2
  localSurfaceCubicEval : Subsystem
  BTQadj : Outport  VectorParamsAs1DForOutWhenUnconnected=off
  wires:
  localSurfaceCubicEval/1(Y) -> BTQadj/1
  SPARK/1 -> localSurfaceCubicEval/2(X)
  Param/1 -> localSurfaceCubicEval/1(P)

== system Engine_Lib/Data Driven/MBC Engine Model From Dynamometer Data/MBC Brake Torque/xregtwostage/RF1 ==
  X : Inport
  Code : Subsystem
  hybridRBFEval : Subsystem
  term : Terminator
  Y : Outport  VectorParamsAs1DForOutWhenUnconnected=off
  wires:
  hybridRBFEval/2(J) -> term/1
  hybridRBFEval/1(Y) -> Y/1
  Code/1(XCoded) -> hybridRBFEval/1(X)
  X/1 -> Code/1(XIn)

== system Engine_Lib/Data Driven/MBC Engine Model From Dynamometer Data/MBC Brake Torque/xregtwostage/RF2 ==
  X : Inport
  Code : Subsystem
  hybridRBFEval : Subsystem
  term : Terminator
  Y : Outport  VectorParamsAs1DForOutWhenUnconnected=off
  wires:
  hybridRBFEval/2(J) -> term/1
  hybridRBFEval/1(Y) -> Y/1
  Code/1(XCoded) -> hybridRBFEval/1(X)
  X/1 -> Code/1(XIn)

== system Engine_Lib/Data Driven/MBC Engine Model From Dynamometer Data/MBC Brake Torque/xregtwostage/RF3 ==
  X : Inport
  Code : Subsystem
  hybridRBFEval : Subsystem
  term : Terminator
  Y : Outport  VectorParamsAs1DForOutWhenUnconnected=off
  wires:
  hybridRBFEval/2(J) -> term/1
  hybridRBFEval/1(Y) -> Y/1
  Code/1(XCoded) -> hybridRBFEval/1(X)
  X/1 -> Code/1(XIn)

== system Engine_Lib/Data Driven/MBC Engine Model From Dynamometer Data/MBC Brake Torque/xregtwostage/Reconstruct ==
  Param : Inport
  Constant : Constant  Value=invDG(:)
  Linear Reconstruct : Gain  Gain=invDG  Multiplication=Matrix(K*u)  SaturateOnIntegerOverflow=on  OutDataTypeStr=Inherit: Same as input  ParamDataTypeStr=Inherit: Same as input
  Param Rec : Outport  VectorParamsAs1DForOutWhenUnconnected=off
  h : Outport  Port=2  VectorParamsAs1DForOutWhenUnconnected=off
  wires:
  Linear Reconstruct/1 -> Param Rec/1
  Param/1 -> Linear Reconstruct/1
  Constant/1 -> h/1

== system Engine_Lib/Data Driven/MBC Engine Model From Dynamometer Data/MBC Brake Torque/xregtwostage/Local Model/localSurfaceCubicEval ==
  P : Inport
  X : Inport  Port=2
  Assignment : Assignment  DiagnosticForDimensions=Error  IndexOptions=Index vector (dialog)  Indices=termsin  OutputSizes=[1 1]
  Constant1 : Constant  Value=zeros(1, numterms)
  S-Function : S-Function  FunctionName=mvCubicEvalSFnV2  Parameters=orderM, reorderM, interact  SFunctionModules=mvcubiceval_helper  SFunctionDeploymentMode=off  EnableBusSupport=off
  Y : Outport  VectorParamsAs1DForOutWhenUnconnected=off
  wires:
  S-Function/1 -> Y/1
  X/1 -> S-Function/2
  P/1 -> Assignment/2
  Assignment/1 -> S-Function/1
  Constant1/1 -> Assignment/1

== system Engine_Lib/Data Driven/MBC Engine Model From Dynamometer Data/MBC Brake Torque/xregtwostage/RF1/Code ==
  XIn : Inport
  Mid : Constant  Value=[0 0 0 0 0 ]
  demux : Demux  Outputs=5
      settings: DisplayOption=none
  gain : Gain  Gain=[1 1 1 1 1 ]  SaturateOnIntegerOverflow=on  OutDataTypeStr=Inherit: Same as input  ParamDataTypeStr=Inherit: Same as input
  mux : Mux  Inputs=5
  sum : Sum  Inputs=-+|  InputSameDT=on  SaturateOnIntegerOverflow=on  OutDataTypeStr=Inherit: Same as first input
  XCoded : Outport  VectorParamsAs1DForOutWhenUnconnected=off
  wires:
  gain/1 -> XCoded/1
  sum/1 -> gain/1
  mux/1 -> sum/2
  XIn/1 -> demux/1
  Mid/1 -> sum/1
  demux/5 -> mux/5
  demux/4 -> mux/4
  demux/3 -> mux/3
  demux/2 -> mux/2
  demux/1 -> mux/1

== system Engine_Lib/Data Driven/MBC Engine Model From Dynamometer Data/MBC Brake Torque/xregtwostage/RF1/hybridRBFEval ==
  X : Inport
  mvCubicEval : Subsystem
  rbfwendlandEval : Subsystem  mask{NumTerms=WendlandNumTerms, E=exponent, P=polyTerms, B=beta, S=width, C=center}
      mask prompts: NumTerms "Number of Poylnomial Terms"; E "Exponent"; P "Polynomial Terms"; B "Betas"; S "Widths"; C "Centers"
  sum : Sum  InputSameDT=on  SaturateOnIntegerOverflow=on  OutDataTypeStr=Inherit: Same as first input
  Y : Outport  VectorParamsAs1DForOutWhenUnconnected=off
  J : Outport  Port=2  VectorParamsAs1DForOutWhenUnconnected=off
  wires:
  rbfwendlandEval/2(J) -> J/1
  sum/1 -> Y/1
  rbfwendlandEval/1(Y) -> sum/2
  mvCubicEval/1(Y) -> sum/1
  X/1 -> rbfwendlandEval/1(X), mvCubicEval/1(X)

== system Engine_Lib/Data Driven/MBC Engine Model From Dynamometer Data/MBC Brake Torque/xregtwostage/RF2/Code ==
  XIn : Inport
  Mid : Constant  Value=[0 0 0 0 0 ]
  demux : Demux  Outputs=5
      settings: DisplayOption=none
  gain : Gain  Gain=[1 1 1 1 1 ]  SaturateOnIntegerOverflow=on  OutDataTypeStr=Inherit: Same as input  ParamDataTypeStr=Inherit: Same as input
  mux : Mux  Inputs=5
  sum : Sum  Inputs=-+|  InputSameDT=on  SaturateOnIntegerOverflow=on  OutDataTypeStr=Inherit: Same as first input
  XCoded : Outport  VectorParamsAs1DForOutWhenUnconnected=off
  wires:
  gain/1 -> XCoded/1
  sum/1 -> gain/1
  mux/1 -> sum/2
  XIn/1 -> demux/1
  Mid/1 -> sum/1
  demux/5 -> mux/5
  demux/4 -> mux/4
  demux/3 -> mux/3
  demux/2 -> mux/2
  demux/1 -> mux/1

== system Engine_Lib/Data Driven/MBC Engine Model From Dynamometer Data/MBC Brake Torque/xregtwostage/RF2/hybridRBFEval ==
  X : Inport
  mvCubicEval : Subsystem
  rbfmultiquadricEval : Subsystem  mask{B=beta, S=width, C=center}
      mask prompts: B "Betas"; S "Widths"; C "Centers"
  sum : Sum  InputSameDT=on  SaturateOnIntegerOverflow=on  OutDataTypeStr=Inherit: Same as first input
  Y : Outport  VectorParamsAs1DForOutWhenUnconnected=off
  J : Outport  Port=2  VectorParamsAs1DForOutWhenUnconnected=off
  wires:
  rbfmultiquadricEval/2(J) -> J/1
  sum/1 -> Y/1
  rbfmultiquadricEval/1(Y) -> sum/2
  mvCubicEval/1(Y) -> sum/1
  X/1 -> rbfmultiquadricEval/1(X), mvCubicEval/1(X)

== system Engine_Lib/Data Driven/MBC Engine Model From Dynamometer Data/MBC Brake Torque/xregtwostage/RF3/Code ==
  XIn : Inport
  Mid : Constant  Value=[0 0 0 0 0 ]
  demux : Demux  Outputs=5
      settings: DisplayOption=none
  gain : Gain  Gain=[1 1 1 1 1 ]  SaturateOnIntegerOverflow=on  OutDataTypeStr=Inherit: Same as input  ParamDataTypeStr=Inherit: Same as input
  mux : Mux  Inputs=5
  sum : Sum  Inputs=-+|  InputSameDT=on  SaturateOnIntegerOverflow=on  OutDataTypeStr=Inherit: Same as first input
  XCoded : Outport  VectorParamsAs1DForOutWhenUnconnected=off
  wires:
  gain/1 -> XCoded/1
  sum/1 -> gain/1
  mux/1 -> sum/2
  XIn/1 -> demux/1
  Mid/1 -> sum/1
  demux/5 -> mux/5
  demux/4 -> mux/4
  demux/3 -> mux/3
  demux/2 -> mux/2
  demux/1 -> mux/1

== system Engine_Lib/Data Driven/MBC Engine Model From Dynamometer Data/MBC Brake Torque/xregtwostage/RF3/hybridRBFEval ==
  X : Inport
  mvCubicEval : Subsystem
  rbfmultiquadricEval : Subsystem  mask{B=beta, S=width, C=center}
      mask prompts: B "Betas"; S "Widths"; C "Centers"
  sum : Sum  InputSameDT=on  SaturateOnIntegerOverflow=on  OutDataTypeStr=Inherit: Same as first input
  Y : Outport  VectorParamsAs1DForOutWhenUnconnected=off
  J : Outport  Port=2  VectorParamsAs1DForOutWhenUnconnected=off
  wires:
  rbfmultiquadricEval/2(J) -> J/1
  sum/1 -> Y/1
  rbfmultiquadricEval/1(Y) -> sum/2
  mvCubicEval/1(Y) -> sum/1
  X/1 -> rbfmultiquadricEval/1(X), mvCubicEval/1(X)

== system Engine_Lib/Data Driven/MBC Engine Model From Dynamometer Data/MBC Brake Torque/xregtwostage/RF1/hybridRBFEval/mvCubicEval ==
  X : Inport
  Constant : Constant  Value=coeffs
  S-Function : S-Function  FunctionName=mvCubicEvalSFnV2  Parameters=orderM, reorderM, interact  SFunctionModules=mvcubiceval_helper  SFunctionDeploymentMode=off  EnableBusSupport=off
  Y : Outport  VectorParamsAs1DForOutWhenUnconnected=off
  wires:
  Constant/1 -> S-Function/1
  S-Function/1 -> Y/1
  X/1 -> S-Function/2

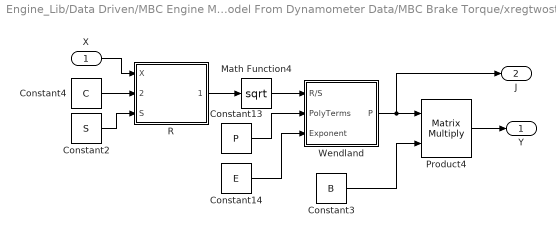
== system Engine_Lib/Data Driven/MBC Engine Model From Dynamometer Data/MBC Brake Torque/xregtwostage/RF1/hybridRBFEval/rbfwendlandEval ==
  X : Inport
  Constant13 : Constant  Value=P
  Constant14 : Constant  Value=E
  Constant2 : Constant  Value=S  VectorParams1D=off
  Constant3 : Constant  Value=B
  Constant4 : Constant  Value=C  VectorParams1D=off
  Math Function4 : Math  Operator=sqrt  SignedPower=on
  Product4 : Product  Multiplication=Matrix(*)  InputSameDT=on  SaturateOnIntegerOverflow=on  OutDataTypeStr=Inherit: Same as first input
  R : Subsystem
  Wendland : Subsystem  mask{NumTerms=NumTerms}
      mask prompts: NumTerms "Number of Polynomial Terms"
  Y : Outport  VectorParamsAs1DForOutWhenUnconnected=off
  J : Outport  Port=2  VectorParamsAs1DForOutWhenUnconnected=off
  wires:
  Constant14/1 -> Wendland/3(Exponent)
  Product4/1 -> Y/1
  Wendland/1(P) -> J/1, Product4/1
  Constant3/1 -> Product4/2
  Math Function4/1 -> Wendland/1(R/S)
  Constant4/1 -> R/2("Centers ")
  X/1 -> R/1(X)
  Constant2/1 -> R/3(S)
  R/1((R/S)^2) -> Math Function4/1
  Constant13/1 -> Wendland/2(PolyTerms)

== system Engine_Lib/Data Driven/MBC Engine Model From Dynamometer Data/MBC Brake Torque/xregtwostage/RF2/hybridRBFEval/mvCubicEval ==
  X : Inport
  Constant : Constant  Value=coeffs
  S-Function : S-Function  FunctionName=mvCubicEvalSFnV2  Parameters=orderM, reorderM, interact  SFunctionModules=mvcubiceval_helper  SFunctionDeploymentMode=off  EnableBusSupport=off
  Y : Outport  VectorParamsAs1DForOutWhenUnconnected=off
  wires:
  Constant/1 -> S-Function/1
  S-Function/1 -> Y/1
  X/1 -> S-Function/2

== system Engine_Lib/Data Driven/MBC Engine Model From Dynamometer Data/MBC Brake Torque/xregtwostage/RF2/hybridRBFEval/rbfmultiquadricEval ==
  X : Inport
  Constant2 : Constant  Value=S  VectorParams1D=off
  Constant3 : Constant  Value=B
  Constant4 : Constant  Value=C  VectorParams1D=off
  MqGlobalWidth : Subsystem
  Product4 : Product  Multiplication=Matrix(*)  InputSameDT=on  SaturateOnIntegerOverflow=on  OutDataTypeStr=Inherit: Same as first input
  R : Subsystem
  Y : Outport  VectorParamsAs1DForOutWhenUnconnected=off
  J : Outport  Port=2  VectorParamsAs1DForOutWhenUnconnected=off
  wires:
  R/1((R/S)^2) -> MqGlobalWidth/1((R/S)^2)
  Constant2/1 -> R/3(S), MqGlobalWidth/2(S)
  X/1 -> R/1(X)
  Constant4/1 -> R/2("Centers ")
  Product4/1 -> Y/1
  MqGlobalWidth/1(P) -> Product4/1, J/1
  Constant3/1 -> Product4/2

== system Engine_Lib/Data Driven/MBC Engine Model From Dynamometer Data/MBC Brake Torque/xregtwostage/RF3/hybridRBFEval/mvCubicEval ==
  X : Inport
  Constant : Constant  Value=coeffs
  S-Function : S-Function  FunctionName=mvCubicEvalSFnV2  Parameters=orderM, reorderM, interact  SFunctionModules=mvcubiceval_helper  SFunctionDeploymentMode=off  EnableBusSupport=off
  Y : Outport  VectorParamsAs1DForOutWhenUnconnected=off
  wires:
  Constant/1 -> S-Function/1
  S-Function/1 -> Y/1
  X/1 -> S-Function/2

== system Engine_Lib/Data Driven/MBC Engine Model From Dynamometer Data/MBC Brake Torque/xregtwostage/RF3/hybridRBFEval/rbfmultiquadricEval ==
  X : Inport
  Constant2 : Constant  Value=S  VectorParams1D=off
  Constant3 : Constant  Value=B
  Constant4 : Constant  Value=C  VectorParams1D=off
  MqGlobalWidth : Subsystem
  Product4 : Product  Multiplication=Matrix(*)  InputSameDT=on  SaturateOnIntegerOverflow=on  OutDataTypeStr=Inherit: Same as first input
  R : Subsystem
  Y : Outport  VectorParamsAs1DForOutWhenUnconnected=off
  J : Outport  Port=2  VectorParamsAs1DForOutWhenUnconnected=off
  wires:
  R/1((R/S)^2) -> MqGlobalWidth/1((R/S)^2)
  Constant2/1 -> R/3(S), MqGlobalWidth/2(S)
  X/1 -> R/1(X)
  Constant4/1 -> R/2("Centers ")
  Product4/1 -> Y/1
  MqGlobalWidth/1(P) -> Product4/1, J/1
  Constant3/1 -> Product4/2

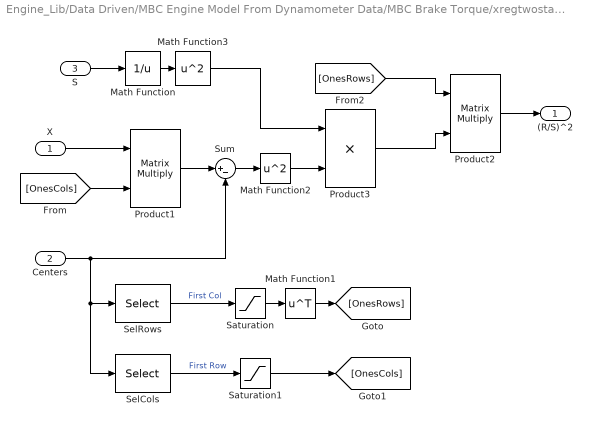
== system Engine_Lib/Data Driven/MBC Engine Model From Dynamometer Data/MBC Brake Torque/xregtwostage/RF1/hybridRBFEval/rbfwendlandEval/R ==
  X : Inport
  "Centers " : Inport  Port=2
  S : Inport  Port=3
  Math Function : Math  Operator=reciprocal  SignedPower=on
  Math Function1 : Math  Operator=transpose  SignedPower=on
  Math Function2 : Math  Operator=square  SignedPower=on
  Math Function3 : Math  Operator=square  SignedPower=on
  Product1 : Product  Multiplication=Matrix(*)  InputSameDT=on  SaturateOnIntegerOverflow=on  OutDataTypeStr=Inherit: Same as first input
  Product2 : Product  Multiplication=Matrix(*)  InputSameDT=on  SaturateOnIntegerOverflow=on  OutDataTypeStr=Inherit: Same as first input
  Product3 : Product  InputSameDT=on  SaturateOnIntegerOverflow=on  OutDataTypeStr=Inherit: Same as first input
  Saturation : Saturate  UpperLimit=1  LowerLimit=1
  Saturation1 : Saturate  UpperLimit=1  LowerLimit=1
  SelCols : Selector  NumberOfDimensions=2  InputPortWidth=3  IndexOptions=Index vector (dialog),Select all  Indices=1,-1  OutputSizes=1
  SelRows : Selector  NumberOfDimensions=2  InputPortWidth=3  IndexOptions=Select all,Index vector (dialog)  Indices=-1,1  OutputSizes=1
  Sum : Sum  Inputs=|+-  InputSameDT=on  SaturateOnIntegerOverflow=on  OutDataTypeStr=Inherit: Same as first input
  (R/S)^2 : Outport  VectorParamsAs1DForOutWhenUnconnected=off
  wires:
  Math Function2/1 -> Product3/2
  Sum/1 -> Math Function2/1
  Product1/1 -> Sum/1
  X/1 -> Product1/1
  [OnesCols] -> Product1/2
  Math Function1/1 -> [OnesRows]
  SelRows/1 -> Saturation/1  "First Col"
  "Centers "/1 -> Sum/2, SelRows/1, SelCols/1
  S/1 -> Math Function/1
  Math Function/1 -> Math Function3/1
  Saturation/1 -> Math Function1/1
  SelCols/1 -> Saturation1/1  "First Row"
  Saturation1/1 -> [OnesCols]
  Math Function3/1 -> Product3/1
  Product3/1 -> Product2/2
  Product2/1 -> (R/S)^2/1
  [OnesRows] -> Product2/1
